simulink model "IEEE13_DVR_DSTATCOM_PV_Wind"  (R2022a)
settings: Solver=ode4  StartTime=0.0  StopTime=1.0  FixedStep=Ts  MaxStep=1e-4  RelTol=1e-4
InitFcn:
  | a=1; % Loading Factor
  | Ts=50e-6;
  | % phase to sequence conversion of RXB matrices
  | c=1*exp(sqrt(-1)*(120*pi/180));
  | T=[1 1 1;1 c*c c;1 c c*c];
  | Tinv=1/3*[1 1 1;1 c c*c;1 c*c c];
  | 
  | % Simulation data for the IEEE 13 Node Test Feeder model
  | mi2km = 1.60934;%  miles to km conversion
  | ft2km = 0.0003048; % feet to km conversion
  | ms2F = 1*1e-6/(2*pi*60);% microsiemens to Farads conversion
  | 
  | 
  | %% Configuration 601
  | % Series Resitance and Reactance - ohm/mile
  | R_601 = [0.3465 0.1560 0.1580;0.1560 0.3375 0.1535;0.1580 0.1535 0.3414];
  | X_601 = [1.1079 0.5017 0.4236;0.5017 1.0478 0.3849;0.4236 0.3849 1.0348];
  | % charging susceptance - microsiemens/mile
  | B_601 = [6.2998 -1.9958 -1.2595;-1.9958 5.9597 -0.7417;-1.2595 -0.7417 5.6386];
  | 
  | R_601 = R_601/mi2km;
  | Rseq=Tinv*R_601*T;
  | R1_601=Rseq(2,2);R0_601=Rseq(1,1);
  | 
  | L_601 = (X_601/(2*pi*60))/mi2km;
  | Lseq=Tinv*L_601*T;
  | L1_601=Lseq(2,2);L0_601=Lseq(1,1);
  | 
  | C_601 =(B_601*ms2F)/mi2km;
  | Cseq=Tinv*C_601*T;
  | C1_601=Cseq(2,2);C0_601=Cseq(1,1);
  | 
  | %% Configuration 602 - series reactance - ohm/mile
  | R_602 = [0.7526 0.1580 0.1560;0.1580 0.7475 0.1535;0.1560 0.1535 0.7436];
  | X_602 = [1.1814 0.4236 0.5017;0.4236 1.1983 0.3849;0.5017 0.3849 1.2112];
  | % charging susceptance - microsiemens/mile
  | B_602 = [5.6990 -1.0817 -1.6905;-1.0817 5.1795 -0.6588;-1.6905 -0.6588 5.4246];
  | 
  | R_602 = R_602/mi2km;
  | Rseq=Tinv*R_602*T;
  | R1_602=Rseq(2,2);R0_602=Rseq(1,1);
  | 
  | L_602 = (X_602/(2*pi*60))/mi2km;
  | Lseq=Tinv*L_602*T;
  | L1_602=Lseq(2,2);L0_602=Lseq(1,1);
  | 
  | C_602 =(B_602*ms2F)/mi2km;
  | Cseq=Tinv*C_602*T;
  | C1_602=Cseq(2,2);C0_602=Cseq(1,1);
  | %% Configuration 603 - series reactance - ohm/mile
  | R_603 = [0 0 0;0 1.3294 0.2066;0 0.2066 1.3238];
  | X_603 = [0 0 0;0 1.3471 0.4591;0 0.4591 1.3569];
  | % charging susceptance - microsiemens/mile
  | B_603 = [0 0 0;0 4.7097 -0.8999;0 -0.8999 4.6658];
  | 
  | % convert for SPS
  | R_603 = R_603/mi2km;
  | Rseq=Tinv*R_603*T;
  | R1_603=Rseq(2,2);R0_603=Rseq(1,1);
  | 
  | L_603 = (X_603/(2*pi*60))/mi2km;
  | Lseq=Tinv*L_603*T;
  | L1_603=Lseq(2,2);L0_603=Lseq(1,1);
  | 
  | C_603 =(B_603*ms2F)/mi2km;
  | Cseq=Tinv*C_603*T;
  | C1_603=Cseq(2,2);C0_603=Cseq(1,1);
  | %% Configuration 604 - series reactance - ohm/mile
  | R_604 = [1.3238 0 0.2066;0 0 0;0.2066 0 1.3294];
  | X_604 = [1.3569 0 0.4591;0 0 0;0.4591 0 1.3471];
  | % charging susceptance - microsiemens/mile
  | B_604 = [4.6658 0 -0.8999;0 0 0;-0.8999 0 4.7097];
  | R_604 = R_604/mi2km;
  | Rseq=Tinv*R_604*T;
  | R1_604=Rseq(2,2);R0_604=Rseq(1,1);
  | 
  | L_604 = (X_604/(2*pi*60))/mi2km;
  | Lseq=Tinv*L_604*T;
  | L1_604=Lseq(2,2);L0_604=Lseq(1,1);
  | 
  | C_604 =(B_604*ms2F)/mi2km;
  | Cseq=Tinv*C_604*T;
  | C1_604=Cseq(2,2);C0_604=Cseq(1,1);
  | %% Configuration 605 - series reactance - ohm/mile
  | R_605 = [0 0 0;0 0 0;0 0 1.3292];
  | X_605 = [0 0 0;0 0 0;0 0 1.3475];
  | % charging susceptance - microsiemens/mile
  | B_605 = [0 0 0;0 0 0;0 0 4.5193];
  | R_605 = R_605/mi2km;
  | Rseq=Tinv*R_605*T;
  | R1_605=Rseq(2,2);R0_605=Rseq(1,1);
  | 
  | L_605 = (X_605/(2*pi*60))/mi2km;
  | Lseq=Tinv*L_605*T;
  | L1_605=Lseq(2,2);L0_605=Lseq(1,1);
  | 
  | C_605 =(B_605*ms2F)/mi2km;
  | Cseq=Tinv*C_605*T;
  | C1_605=Cseq(2,2);C0_605=Cseq(1,1);
  | %% Configuration 606 - series reactance - ohm/mile
  | R_606 = [0.7982 0.3192 0.2849;0.3192 0.7891 0.3192;0.2849 0.3192 0.7982];
  | X_606 = [0.4463 0.0328 0.0143;0.0328 0.4041 0.0328;0.0143 0.0328 0.4463];
  | % charging susceptance - microsiemens/mile
  | B_606 = [96.8897 -1e-6 -1e-6;-1e-6 96.8897 -1e-6;-1e-6 -1e-6 96.8897];
  | R_606 = R_606/mi2km;
  | Rseq=Tinv*R_606*T;
  | R1_606=Rseq(2,2);R0_606=Rseq(1,1);
  | 
  | L_606 = (X_606/(2*pi*60))/mi2km;
  | Lseq=Tinv*L_606*T;
  | L1_606=Lseq(2,2);L0_606=Lseq(1,1);
  | 
  | C_606 =(B_606*ms2F)/mi2km;
  | Cseq=Tinv*C_606*T;
  | C1_606=Cseq(2,2);C0_606=Cseq(1,1);
  | %% Configuration 607 - series reactance - ohm/mile
  | R_607 = [1.3425 0 0;0 0 0;0 0 0];
  | X_607 = [0.5124 0 0;0 0 0;0 0 0];
  | % charging susceptance - microsiemens/mile
  | B_607 = [88.9912 0 0;0 0 0;0 0 0];
  | R_607 = R_607/mi2km;
  | Rseq=Tinv*R_607*T;
  | R1_607=Rseq(2,2);R0_607=Rseq(1,1);
  | 
  | L_607 = (X_607/(2*pi*60))/mi2km;
  | Lseq=Tinv*L_607*T;
  | L1_607=Lseq(2,2);L0_607=Lseq(1,1);
  | 
  | C_607 =(B_607*ms2F)/mi2km;
  | Cseq=Tinv*C_607*T;
  | C1_607=Cseq(2,2);C0_607=Cseq(1,1);
undefined symbols (not defined in the file): find_system
libraries: spsGroundLib x48, spsSeriesRLCBranchLib x46, spsThreePhaseVIMeasurementLib x19, spsControlledVoltageSourceLib x15, spsThreePhaseSeriesRLCLoadLib x7, spsRMSLib x7, spsThreePhaseBreakerLib x6, spsVoltageMeasurementLib x6, spsOnDelayLib x6, spsThreePhasePISectionLineLib x5, spsSeriesRLCLoadLib x5, spsMutualInductanceLib x4
(part 1 of 4)
settings Model: ARTEMISmethode_block_infos=$$__separator__$$pi34variableloadwith3PV/ARTEMIS Guide$$__separator__$$  Creator=Arun  LastModifiedBy=subas
settings SolverCC: ShapePreserveControl=EnableAll  AlgebraicLoopSolver=TrustRegion  SolverResetMethod=Robust
settings DataIOCC: ReturnWorkspaceOutputs=off
settings DebuggingCC: ArithmeticOperatorsInVariantConditions=warning
settings SFSimCC: SimUseLocalCustomCode=off  CustomCodeUndefinedFunction=UseInterfaceOnly
settings RTWCC: RTWUseLocalCustomCode=off
settings CodeAppCC: StateflowObjectComments=on
settings SimscapeCC: SimscapeNormalizeSystem=off

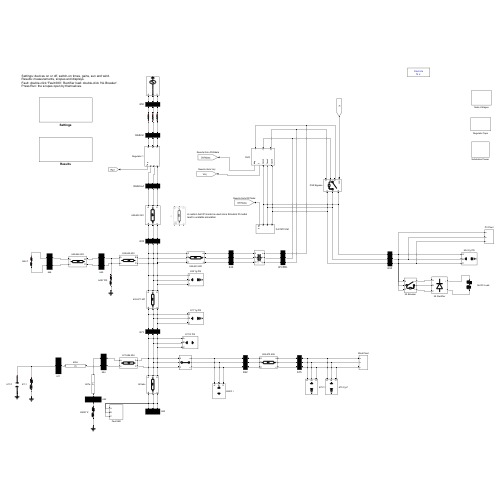
[thumbnail: Simulink's stored preview of the top-level diagram]
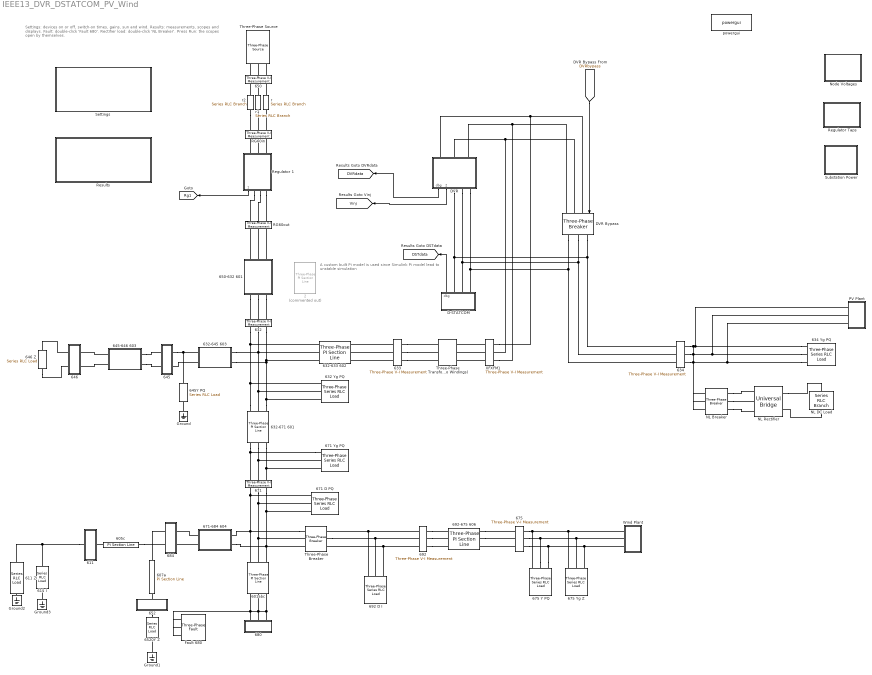
== system IEEE13_DVR_DSTATCOM_PV_Wind ==
  note: A custom built Pi model is used since Simulink Pi model
      | lead to unstable simulation
  note: Settings: devices on or off, switch-on times, gains, sun and wind.
      | Results: measurements, scopes and displays.
      | Fault: double-click 'Fault 680'. Rectifier load: double-click 'NL Breaker'.
      | Press Run: the scopes open by themselves.
  2 : spsThreePhasePISectionLineLib/Three-Phase PI Section Line  Commented=on  LConnTagsString=a|b|c  RConnTagsString=A|B|C  Length=2000*ft2km  Frequency=60  Resistances=[R1_601 R0_601]  Inductances=[L1_601 L0_601]  Capacitances=[C1_601 C0_601]
  601abc : spsThreePhasePISectionLineLib/Three-Phase PI Section Line  LConnTagsString=a|b|c  RConnTagsString=A|B|C  Length=1000*ft2km  Frequency=60  Resistances=[R1_601 R0_601]  Inductances=[L1_601 L0_601]  Capacitances=[C1_601 C0_601]
  605c : spsPiSectionLineLib/Pi Section Line  LConnTagsString=__new0  RConnTagsString=__new0  Phases=1  PiSections=1  Length=300*ft2km  Frequency=60  Resistance=R1_605  Inductance=L1_605  Capacitance=C1_605  SpecifyConductance=off  Conductance=0  Measurements=None  Measurements2=None
  607a : spsPiSectionLineLib/Pi Section Line  LConnTagsString=__new0  RConnTagsString=__new0  Phases=1  PiSections=1  Length=800*ft2km  Frequency=60  Resistance=R1_607  Inductance=L1_607  Capacitance=C1_607  SpecifyConductance=off  Conductance=0  Measurements=None  Measurements2=None
  611 : Subsystem
  611 I : spsSeriesRLCLoadLib/Series RLC Load  LConnTagsString=a  RConnTagsString=__new0  NominalVoltage=1*2401.78  NominalFrequency=60  ActivePower=170e3*a  InductivePower=80e3*a  CapacitivePower=0  Setx0=off  InitialVoltage=0  SetiL0=off  InitialCurrent=0  Measurements=None  LoadType=constant I
  611 Z : spsSeriesRLCLoadLib/Series RLC Load  LConnTagsString=a  RConnTagsString=__new0  NominalVoltage=2401.78  NominalFrequency=60  ActivePower=0  InductivePower=0  CapacitivePower=100e3*a  Setx0=off  InitialVoltage=0  SetiL0=off  InitialCurrent=0  Measurements=None  LoadType=constant Z
  632 : spsThreePhaseVIMeasurementLib/Three-Phase V-I Measurement  VoltageMeasurement=phase-to-ground  SetLabelV=on  LabelV=V632  Vpu=off  VpuLL=off  CurrentMeasurement=yes  SetLabelI=on  LabelI=I632  Ipu=off  Pbase=100e6  Vbase=24900  OutputType=Complex  PhasorSimulation=off  PSBequivalent=0
  632 Yg PQ : spsThreePhaseSeriesRLCLoadLib/Three-Phase Series RLC Load  LConnTagsString=A|B|C  Configuration=Y (grounded)  NominalVoltage=[ 1.021 1.042 1.0174]*2401.78  Vabc=[ 1 1 1]*2401.78  Vabcp=[1e3 1e3 1e3]  NominalFrequency=60  UnbalancedPower=on  ActivePower="[17 66  117]*1e3/2"  InductivePower="[10 38  68]*1e3/2"  CapacitivePower=100  Pabc="[17 66  117]*1e3/2*a"  QLabc="[10 38  68]*1e3/2*a"  QCabc=[0 0 0]  Pabcp=[10e3 9e3 11e3]  QLabcp=[100 90 110]  QCabcp=[100 90 110]  Measurements=None  LoadType=constant PQ
  632-633 602 : spsThreePhasePISectionLineLib/Three-Phase PI Section Line  LConnTagsString=a|b|c  RConnTagsString=A|B|C  Length=500*ft2km  Frequency=60  Resistances=[R1_602 R0_602]  Inductances=[L1_602 L0_602]  Capacitances=[C1_602 C0_602]
  632-645 603 : Subsystem  mask(Two-Phase PI Section Block){Rl=R_603, Ll=L_603, Cl=C_603, L=500*ft2km}
      mask prompts: Rl "Resistance per unit Length(Ohm/Km)[3x3 matrix]"; Ll "Inductance per unit Length(H/Km)[3x3 matrix]"; Cl "Capacitance per unit Length(F/Km)[3x3 matrix"; L "Length (Km)"
      mask help: This block models a two-phase transmission line with a single PI section.
      mask init:
      | W = sign(sum(abs(Rl)));
      | s = find(W==1);%Identify non zero rows and columns
      | 
      | Rt =Rl(s,s);
      | Rl= Rt;
      | Lt =Ll(s,s);
      | Ll= Lt;
      | Ct =Cl(s,s);
      | Cl= Ct;
      mask Display:
      | color('black')
      | plot(0,0,100,100,[20,20,80,80,90,80,80,20,20,10],[50,40,40,50,50,50,61,61,50,50],[56,39],[55,55],[44,44],[44,55],[53,50,50],[44,48,55])
      | color('black')
      | port_label('RConn', 1, 'b')
      | port_label('RConn', 2, 'c')
      | port_label('LConn', 1, 'B')
      | port_label('LConn', 2, 'C')
  632-671 601 : spsThreePhasePISectionLineLib/Three-Phase PI Section Line  LConnTagsString=a|b|c  RConnTagsString=A|B|C  Length=2000*ft2km  Frequency=60  Resistances=[R1_601 R0_601]  Inductances=[L1_601 L0_601]  Capacitances=[C1_601 C0_601]
  633 : spsThreePhaseVIMeasurementLib/Three-Phase V-I Measurement  VoltageMeasurement=phase-to-ground  SetLabelV=on  LabelV=V633  Vpu=off  VpuLL=off  CurrentMeasurement=no  SetLabelI=on  LabelI=I634  Ipu=off  Pbase=100e6  Vbase=24900  OutputType=Complex  PhasorSimulation=off  PSBequivalent=0
  634 : spsThreePhaseVIMeasurementLib/Three-Phase V-I Measurement  VoltageMeasurement=phase-to-ground  SetLabelV=on  LabelV=V634  Vpu=off  VpuLL=off  CurrentMeasurement=yes  SetLabelI=on  LabelI=I634  Ipu=off  Pbase=100e6  Vbase=24900  OutputType=Complex  PhasorSimulation=off  PSBequivalent=0
  634 Yg PQ : spsThreePhaseSeriesRLCLoadLib/Three-Phase Series RLC Load  LConnTagsString=A|B|C  Configuration=Y (grounded)  NominalVoltage=[ 1.021 1.042 1.0174]*2401.78  Vabc=[1 1 1]*277.128  Vabcp=[1e3 1e3 1e3]  NominalFrequency=60  UnbalancedPower=on  ActivePower="[17 66  117]*1e3/2"  InductivePower="[10 38  68]*1e3/2"  CapacitivePower=100  Pabc=[160 120 120]*1e3*a  QLabc=[110 90 90]*1e3*a  QCabc=[0 0 0]  Pabcp=[10e3 9e3 11e3]  QLabcp=[100 90 110]  QCabcp=[100 90 110]  Measurements=None  LoadType=constant PQ
  645 : Subsystem
  645-646 603 : Subsystem  mask(Two-Phase PI Section Block){Rl=R_603, Ll=L_603, Cl=C_603, L=300*ft2km}
      mask prompts: Rl "Resistance per unit Length(Ohm/Km)[3x3 matrix]"; Ll "Inductance per unit Length(H/Km)[3x3 matrix]"; Cl "Capacitance per unit Length(F/Km)[3x3 matrix"; L "Length (Km)"
      mask help: This block models a two-phase transmission line with a single PI section.
      mask init:
      | W = sign(sum(abs(Rl)));
      | s = find(W==1);%Identify non zero rows and columns
      | 
      | Rt =Rl(s,s);
      | Rl= Rt;
      | Lt =Ll(s,s);
      | Ll= Lt;
      | Ct =Cl(s,s);
      | Cl= Ct;
      mask Display:
      | color('black')
      | plot(0,0,100,100,[20,20,80,80,90,80,80,20,20,10],[50,40,40,50,50,50,61,61,50,50],[56,39],[55,55],[44,44],[44,55],[53,50,50],[44,48,55])
      | color('black')
      | port_label('RConn', 1, 'b')
      | port_label('RConn', 2, 'c')
      | port_label('LConn', 1, 'B')
      | port_label('LConn', 2, 'C')
  645Y PQ : spsSeriesRLCLoadLib/Series RLC Load  LConnTagsString=a  RConnTagsString=__new0  NominalVoltage=1*2401.78  NominalFrequency=60  ActivePower=170e3*a  InductivePower=125e3*a  CapacitivePower=0  Setx0=off  InitialVoltage=0  SetiL0=off  InitialCurrent=0  Measurements=None  LoadType=constant PQ
  646 : Subsystem
  646 Z : spsSeriesRLCLoadLib/Series RLC Load  LConnTagsString=a  RConnTagsString=__new0  NominalVoltage=4160  NominalFrequency=60  ActivePower=230e3*a  InductivePower=132e3*a  CapacitivePower=0  Setx0=off  InitialVoltage=0  SetiL0=off  InitialCurrent=0  Measurements=None  LoadType=constant Z
  650 : spsThreePhaseVIMeasurementLib/Three-Phase V-I Measurement  VoltageMeasurement=phase-to-ground  SetLabelV=on  LabelV=V650  Vpu=off  VpuLL=off  CurrentMeasurement=yes  SetLabelI=on  LabelI=I650  Ipu=off  Pbase=100e6  Vbase=24900  OutputType=Complex  PhasorSimulation=off  PSBequivalent=0
  650-632 601 : Subsystem  mask(Three-Phase PI Section Block){Rl=R_601, Ll=L_601, Cl=C_601, L=2000*ft2km}
      mask prompts: Rl "Resistance per unit Length(Ohm/Km)[3x3 matrix]"; Ll "Inductance per unit Length(H/Km)[3x3 matrix]"; Cl "Capacitance per unit Length(F/Km)[3x3 matrix]"; L "Length (Km)"
      mask help: This block models a three-phase transmission line with a single PI section.
      mask Display:
      | color('black')
      | plot(0,0,100,100,[20,20,80,80,90,80,80,20,20,10],[50,40,40,50,50,50,61,61,50,50],[56,39],[55,55],[44,44],[44,55],[53,50,50],[44,48,55])
      | color('black')
      | port_label('RConn', 1, 'a')
      | port_label('RConn', 2, 'b')
      | port_label('RConn', 3, 'c')
      | port_label('LConn', 1, 'A')
      | port_label('LConn', 2, 'B')
      | port_label('LConn', 3, 'C')
  652 : Subsystem
  6520Y Z : spsSeriesRLCLoadLib/Series RLC Load  LConnTagsString=a  RConnTagsString=__new0  NominalVoltage=1.0*2401.78  NominalFrequency=60  ActivePower=128e3*a  InductivePower=86e3*a  CapacitivePower=0  Setx0=off  InitialVoltage=0  SetiL0=off  InitialCurrent=0  Measurements=None  LoadType=constant Z
  671 : spsThreePhaseVIMeasurementLib/Three-Phase V-I Measurement  VoltageMeasurement=phase-to-ground  SetLabelV=on  LabelV=V671  Vpu=off  VpuLL=off  CurrentMeasurement=no  SetLabelI=on  LabelI=I634  Ipu=off  Pbase=100e6  Vbase=24900  OutputType=Complex  PhasorSimulation=off  PSBequivalent=0
  671 D PQ : spsThreePhaseSeriesRLCLoadLib/Three-Phase Series RLC Load  LConnTagsString=A|B|C  Configuration=Delta  NominalVoltage=[ 1.021 1.042 1.0174]*2401.78  Vabc=[ 1.73773 1.77224 1.71484]*2401.78  Vabcp=[ 1 1 1]*4160  NominalFrequency=60  UnbalancedPower=on  ActivePower="[17 66  117]*1e3/2"  InductivePower="[10 38  68]*1e3/2"  CapacitivePower=100  Pabc=[385 385 385 ]*1e3  QLabc=[220 220 220]*1e3  QCabc=[0 0 0]  Pabcp=[385 385 385 ]*1e3*a  QLabcp=[220 220 220]*1e3*a  QCabcp="[0  0  0]"  Measurements=Branch voltages and currents  LoadType=constant PQ
  671 Yg PQ : spsThreePhaseSeriesRLCLoadLib/Three-Phase Series RLC Load  LConnTagsString=A|B|C  Configuration=Y (grounded)  NominalVoltage=[ 1.021 1.042 1.0174]*2401.78  Vabc=[ 1 1 1]*2401.78  Vabcp=[1e3 1e3 1e3]  NominalFrequency=60  UnbalancedPower=on  ActivePower="[17 66  117]*1e3/2"  InductivePower="[10 38  68]*1e3/2"  CapacitivePower=100  Pabc="[17 66  117]*1e3/2*a"  QLabc="[10 38  68]*1e3/2*a"  QCabc=[0 0 0]  Pabcp=[10e3 9e3 11e3]  QLabcp=[100 90 110]  QCabcp=[100 90 110]  Measurements=None  LoadType=constant PQ
  671-684 604 : Subsystem  mask(Two-Phase PI Section Block){Rl=R_604, Ll=L_604, Cl=C_604, L=300*ft2km}
      mask prompts: Rl "Resistance per unit Length(Ohm/Km)[3x3 matrix]"; Ll "Inductance per unit Length(H/Km)[3x3 matrix]"; Cl "Capacitance per unit Length(F/Km)[3x3 matrix"; L "Length (Km)"
      mask help: This block models a two-phase transmission line with a single PI section.
      mask init:
      | W = sign(sum(abs(Rl)));
      | s = find(W==1);%Identify non zero rows and columns
      | 
      | Rt =Rl(s,s);
      | Rl= Rt;
      | Lt =Ll(s,s);
      | Ll= Lt;
      | Ct =Cl(s,s);
      | Cl= Ct;
      mask Display:
      | color('black')
      | plot(0,0,100,100,[20,20,80,80,90,80,80,20,20,10],[50,40,40,50,50,50,61,61,50,50],[56,39],[55,55],[44,44],[44,55],[53,50,50],[44,48,55])
      | color('black')
      | port_label('RConn', 1, 'a')
      | port_label('RConn', 2, 'c')
      | port_label('LConn', 1, 'A')
      | port_label('LConn', 2, 'C')
  675 : spsThreePhaseVIMeasurementLib/Three-Phase V-I Measurement  VoltageMeasurement=phase-to-ground  SetLabelV=on  LabelV=V675  Vpu=off  VpuLL=off  CurrentMeasurement=no  SetLabelI=on  LabelI=I634  Ipu=off  Pbase=100e6  Vbase=24900  OutputType=Complex  PhasorSimulation=off  PSBequivalent=0
  675 Y PQ : spsThreePhaseSeriesRLCLoadLib/Three-Phase Series RLC Load  LConnTagsString=A|B|C  Configuration=Y (grounded)  NominalVoltage=[ 1.021 1.042 1.0174]*2401.78  Vabc=[ 1 1 1]*2401.78  Vabcp=[1e3 1e3 1e3]  NominalFrequency=60  UnbalancedPower=on  ActivePower="[17 66  117]*1e3/2"  InductivePower="[10 38  68]*1e3/2"  CapacitivePower=100  Pabc="[485  68  290]*1e3*a"  QLabc="[190  60  212]*1e3*a"  QCabc=[0 0 0]  Pabcp=[10e3 9e3 11e3]  QLabcp=[100 90 110]  QCabcp=[100 90 110]  Measurements=Branch voltages and currents  LoadType=constant PQ
  675 Yg Z : spsThreePhaseSeriesRLCLoadLib/Three-Phase Series RLC Load  LConnTagsString=A|B|C  Configuration=Y (grounded)  NominalVoltage=[ 1.021 1.042 1.0174]*2401.78  Vabc=[ 1.0 1.0 1.0]*2401.78  Vabcp=[1e3 1e3 1e3]  NominalFrequency=60  UnbalancedPower=on  ActivePower="[17 66  117]*1e3/2"  InductivePower="[10 38  68]*1e3/2"  CapacitivePower=100  Pabc=[0 0 0]  QLabc=[0 0 0]  QCabc=[200 200 200]*1e3*a  Pabcp=[10e3 9e3 11e3]  QLabcp=[100 90 110]  QCabcp=[100 90 110]  Measurements=None  LoadType=constant Z
  680 : Subsystem
  684 : Subsystem
  692 : spsThreePhaseVIMeasurementLib/Three-Phase V-I Measurement  VoltageMeasurement=phase-to-ground  SetLabelV=on  LabelV=V692  Vpu=off  VpuLL=off  CurrentMeasurement=no  SetLabelI=on  LabelI=I634  Ipu=off  Pbase=100e6  Vbase=24900  OutputType=Complex  PhasorSimulation=off  PSBequivalent=0
  692 D I : spsThreePhaseSeriesRLCLoadLib/Three-Phase Series RLC Load  LConnTagsString=A|B|C  Configuration=Delta  NominalVoltage=[ 1.021 1.042 1.0174]*2401.78  Vabc=[ 1.73488 1.75203 1.72341]*2401.78  Vabcp=[ 1.0 1.0 1.0]*4160  NominalFrequency=60  UnbalancedPower=on  ActivePower="[17 66  117]*1e3/2"  InductivePower="[10 38  68]*1e3/2"  CapacitivePower=100  Pabc="[17 66  117]*1e3/2"  QLabc="[10 38  68]*1e3/2"  QCabc=[0 0 0]  Pabcp=[1e-3 1e-3 170 ]*1e3*a  QLabcp=[0 0 151]*1e3*a  QCabcp="[0  0  0]"  Measurements=Branch voltages and currents  LoadType=constant Z
  692-675 606 : spsThreePhasePISectionLineLib/Three-Phase PI Section Line  LConnTagsString=a|b|c  RConnTagsString=A|B|C  Length=500*ft2km  Frequency=60  Resistances=[R1_606 R0_606]  Inductances=[L1_606 L0_606]  Capacitances=[C1_606 C0_606]
  D-STATCOM : Subsystem
  DVR : Subsystem
  DVR Bypass : spsThreePhaseBreakerLib/Three-Phase Breaker  InitialState=open  SwitchA=on  SwitchB=on  SwitchC=on  SwitchTimes="[1/60  5/60]"  External=on  BreakerResistance=1e-3  SnubberResistance=1e6  SnubberCapacitance=inf  Measurements=None
  Fault 680 : spsThreePhaseFaultLib/Three-Phase Fault  InitialStates=0  FaultA=on  FaultB=off  FaultC=off  GroundFault=on  SwitchTimes=[0.6 0.8]  External=off  SwitchStatus=NaN  FaultResistance=0.01  GroundResistance=0.01  SnubberResistance=1e6  SnubberCapacitance=inf  Measurements=None
  Ground{,1..3} (4 alike) : spsGroundLib/Ground  LConnTagsString=a
  NL Breaker : spsThreePhaseBreakerLib/Three-Phase Breaker  InitialState=open  SwitchA=on  SwitchB=on  SwitchC=on  SwitchTimes=[0.3]  External=off  BreakerResistance=0.01  SnubberResistance=1e6  SnubberCapacitance=inf  Measurements=None
  NL DC Load : spsSeriesRLCBranchLib/Series RLC Branch  LConnTagsString=__new0  RConnTagsString=__new0  BranchType=RL  Resistance=4.2  Inductance=5e-3  SetiL0=off  InitialCurrent=0  Capacitance=1e-6  Setx0=off  InitialVoltage=0  Measurements=None
  NL Rectifier : spsUniversalBridgeLib/Universal Bridge  Arms=3  SnubberResistance=1e5  SnubberCapacitance=inf  Device=Diodes  Ron=1e-3  Lon=0  ForwardVoltages="[  0  0  ]"  ForwardVoltage=0  GTOparameters=[ 10e-6 , 20e-6 ]  IGBTparameters=[ 1e-6 , 2e-6 ]  Measurements=None  Measurements_2=None  converterType=Rectifier
  Node Voltages : Subsystem
  PV Plant : Subsystem
  RG60in : spsThreePhaseVIMeasurementLib/Three-Phase V-I Measurement  VoltageMeasurement=phase-to-ground  SetLabelV=on  LabelV=RG60in  Vpu=off  VpuLL=off  CurrentMeasurement=yes  SetLabelI=on  LabelI=IRG60in  Ipu=off  Pbase=100e6  Vbase=24900  OutputType=Complex  PhasorSimulation=off  PSBequivalent=0
  RG60out : spsThreePhaseVIMeasurementLib/Three-Phase V-I Measurement  VoltageMeasurement=phase-to-ground  SetLabelV=on  LabelV=RG60out  Vpu=off  VpuLL=off  CurrentMeasurement=yes  SetLabelI=on  LabelI=IRG60out  Ipu=off  Pbase=100e6  Vbase=24900  OutputType=Complex  PhasorSimulation=off  PSBequivalent=0
  Regulator 1 : Subsystem
  "Regulator Taps " : Subsystem
  Results : Subsystem
  Settings : Subsystem
  Substation Power : Subsystem
  Three-Phase Transformer (Two Windings) : spsThreePhaseTransformerTwoWindingsLib/Three-Phase Transformer (Two Windings)  Winding1Connection=Yg  Winding2Connection=Yg  CoreType=Three single-phase transformers  SetSaturation=off  Hysteresis=off  DataFile='hysteresis'  SetInitialFlux=off  Measurements=None  UNITS=pu  NominalPower=[ 500e3 , 60 ]  Winding1=[4160 0.011 0.02]  Winding2=[480 0 0]  Rm=500  Lm=500  L0=0.5  Saturation=[ 0,0 ; 0.0024,1.2 ; 1.0,1.52 ]  InitialFluxes=[ 0.8 , -0.8 , 0.7 ]  BreakLoop=off  DiscreteSolver=Trapezoidal iterative  DataType=off  TransfoNumber=1
  Three-Phase Breaker : spsThreePhaseBreakerLib/Three-Phase Breaker  InitialState=closed  SwitchA=off  SwitchB=off  SwitchC=off  SwitchTimes=[0.5 ]  External=off  BreakerResistance=0.0001  SnubberResistance=inf  SnubberCapacitance=0  Measurements=None
  Three-Phase Source : spsThreePhaseSourceLib/Three-Phase Source  InternalConnection=Yg  VoltagePhases=on  Voltage=25e3  PhaseAngle=0  Voltage_phases=[ 1.0 1.0 1.0]*2401.78  PhaseAngles_phases=[0 -120 120]  Frequency=60  NonIdealSource=off  SpecifyImpedance=off  Resistance=.001  Inductance=16.58e-6  ShortCircuitLevel=100e6  BaseVoltage=4160  XRratio=7  BusType=swing  Pref=10e3  Qref=0  Prefabc=[10e3, 10e3, 10e3]  Qrefabc=[0, 0, 0]  Qmin=-inf  Qmax=inf
  Wind Plant : Subsystem
  XFXFM1 : spsThreePhaseVIMeasurementLib/Three-Phase V-I Measurement  VoltageMeasurement=phase-to-ground  SetLabelV=on  LabelV=XFXFM1  Vpu=off  VpuLL=off  CurrentMeasurement=yes  SetLabelI=on  LabelI=Is634  Ipu=off  Pbase=100e6  Vbase=24900  OutputType=Complex  PhasorSimulation=off  PSBequivalent=0
  powergui : spspowerguiLib/powergui  Priority=1  SimulationMode=Discrete  SampleTime=Ts  frequency=60  Iterations=50  frequencyindice=0  Pbase=100e6  ErrMax=1e-4  UnitsV=kV  UnitsW=MW  buscounter=0  FunctionMessages=off  echomessages=on  EnableUseOfTLC=off  CurrentSourceSwitches=off  DisableSnubberDevices=off  DisableRonSwitches=off  DisableVfSwitches=off  DisplayEquations=off  AutomaticDiscreteSolvers=off  SolverType=Tustin/Backward Euler (TBE)  Interpol=off  ExternalGateDelay=off  methode=off  Ts=0  x0status=blocks  SPID=off  SwTol=0  HookPort=off  NonlinearTolerance=1e-4  nMaxIteration=100  ContinueOnMaxIteration=off  RestoreLinks=warning  ResistiveCurrentMeasurement=off  Frange=[0:2:500]  Ylog=off  Xlog=on  ShowGrid=off  save=off  variable=ZData  structure=0  ZoomFFT=off  StartTime=0.0  cycles=1  DisplayStyle=1  fundamental=60  FreqAxis=off  MaxFrequency=1000  frequencyindicesteady=1  RmsSteady=1  display=off
  r : spsSeriesRLCBranchLib/Series RLC Branch  LConnTagsString=__new0  RConnTagsString=__new0  BranchType=R  Resistance=1e-6  Inductance=1e-6  SetiL0=off  InitialCurrent=0  Capacitance=1e-6  Setx0=off  InitialVoltage=0  Measurements=None
  r1 : spsSeriesRLCBranchLib/Series RLC Branch  LConnTagsString=__new0  RConnTagsString=__new0  BranchType=R  Resistance=1e-6  Inductance=1e-6  SetiL0=off  InitialCurrent=0  Capacitance=1e-6  Setx0=off  InitialVoltage=0  Measurements=None
  r2 : spsSeriesRLCBranchLib/Series RLC Branch  LConnTagsString=__new0  RConnTagsString=__new0  BranchType=R  Resistance=1e-6  Inductance=1e-6  SetiL0=off  InitialCurrent=0  Capacitance=1e-6  Setx0=off  InitialVoltage=0  Measurements=None
  tag scope: DSTdata=global, DVRdata=global, Rg1=global, Vinj=global
  wires:
  Regulator 1/1(Tap) -> [Rg1]
  DVR/1(dbg) -> [DVRdata]
  DVR/2(Out2) -> [Vinj]
  D-STATCOM/1(dbg) -> [DSTdata]
  [DVRbypass] -> DVR Bypass/1
  connections:
  632-645 603/LConn1 -- 632 Yg PQ/LConn2 -- 632-671 601/LConn2 -- 632-633 602/LConn2 -- 632/RConn2
  Three-Phase Breaker/LConn1 -- 671 D PQ/LConn1 -- 671/RConn1 -- 601abc/LConn1 -- 671-684 604/LConn1
  611/LConn1 -- 611 Z/LConn1 -- 611 I/LConn1
  675 Y PQ/LConn2 -- 675 Yg Z/LConn2 -- Wind Plant/RConn2 -- 675/RConn2
  671 Yg PQ/LConn1 -- 671/LConn1 -- 632-671 601/RConn1
  632-671 601/LConn3 -- 632 Yg PQ/LConn3 -- 632/RConn3 -- 632-633 602/LConn3 -- 632-645 603/LConn2
  601abc/LConn2 -- Three-Phase Breaker/LConn2 -- 671 D PQ/LConn2 -- 671/RConn2
  645/RConn1 -- 632-645 603/RConn1 -- 645Y PQ/LConn1
  692/LConn1 -- 692 D I/LConn1 -- Three-Phase Breaker/RConn1
  Wind Plant/RConn1 -- 675 Yg Z/LConn1 -- 675/RConn1 -- 675 Y PQ/LConn1
  671/LConn3 -- 632-671 601/RConn3 -- 671 Yg PQ/LConn3
  671/LConn2 -- 632-671 601/RConn2 -- 671 Yg PQ/LConn2
  632-671 601/LConn1 -- 632 Yg PQ/LConn1 -- 632/RConn1 -- 632-633 602/LConn1
  692/LConn3 -- 692 D I/LConn3 -- Three-Phase Breaker/RConn3
  671-684 604/LConn2 -- 671 D PQ/LConn3 -- 671/RConn3 -- 601abc/LConn3 -- Three-Phase Breaker/LConn3
  675 Y PQ/LConn3 -- 675 Yg Z/LConn3 -- Wind Plant/RConn3 -- 675/RConn3
  692/LConn2 -- 692 D I/LConn2 -- Three-Phase Breaker/RConn2
  684/LConn1 -- 607a/LConn1
  r1/RConn1 -- RG60in/LConn2
  r/RConn1 -- RG60in/LConn3
  645-646 603/RConn2 -- 646/RConn2
  601abc/RConn1 -- 680/RConn1 -- Fault 680/LConn1
  605c/LConn1 -- 684/LConn2
  692/RConn2 -- 692-675 606/LConn2
  646 Z/RConn1 -- 646/LConn2
  650-632 601/RConn1 -- 632/LConn1
  r1/LConn1 -- 650/RConn2
  692-675 606/RConn1 -- 675/LConn1
  675/LConn3 -- 692-675 606/RConn3
  Regulator 1/LConn3 -- RG60in/RConn3
  650-632 601/RConn3 -- 632/LConn3
  652/LConn1 -- 6520Y Z/LConn1
  Ground1/LConn1 -- 6520Y Z/RConn1
  633/LConn1 -- 632-633 602/RConn1
  Regulator 1/RConn2 -- RG60out/LConn2
  633/LConn3 -- 632-633 602/RConn3
  605c/RConn1 -- 611/RConn1
  XFXFM1/LConn2 -- Three-Phase Transformer (Two Windings)/RConn2
  601abc/RConn3 -- 680/RConn3 -- Fault 680/LConn3
  633/RConn2 -- Three-Phase Transformer (Two Windings)/LConn2
  634 Yg PQ/LConn2 -- 634/RConn2 -- NL Breaker/LConn2 -- PV Plant/RConn2
  Ground3/LConn1 -- 611 I/RConn1
  601abc/RConn2 -- 680/RConn2 -- Fault 680/LConn2
  r/LConn1 -- 650/RConn3
  Regulator 1/LConn1 -- RG60in/RConn1
  Regulator 1/RConn3 -- RG60out/LConn3
  Ground/LConn1 -- 645Y PQ/RConn1
  632-645 603/RConn2 -- 645/RConn2
  633/RConn3 -- Three-Phase Transformer (Two Windings)/LConn3
  634 Yg PQ/LConn3 -- 634/RConn3 -- NL Breaker/LConn3 -- PV Plant/RConn3
  r2/RConn1 -- RG60in/LConn1
  692/RConn1 -- 692-675 606/LConn1
  633/RConn1 -- Three-Phase Transformer (Two Windings)/LConn1
  650/LConn3 -- Three-Phase Source/RConn3
  Regulator 1/LConn2 -- RG60in/RConn2
  633/LConn2 -- 632-633 602/RConn2
  645-646 603/RConn1 -- 646/RConn1
  671-684 604/RConn2 -- 684/RConn2
  692/RConn3 -- 692-675 606/LConn3
  652/RConn1 -- 607a/RConn1
  645-646 603/LConn1 -- 645/LConn1
  650-632 601/LConn3 -- RG60out/RConn3
  650-632 601/LConn2 -- RG60out/RConn2
  650/LConn2 -- Three-Phase Source/RConn2
  XFXFM1/LConn3 -- Three-Phase Transformer (Two Windings)/RConn3
  Ground2/LConn1 -- 611 Z/RConn1
  671-684 604/RConn1 -- 684/RConn1
  Regulator 1/RConn1 -- RG60out/LConn1
  692-675 606/RConn2 -- 675/LConn2
  r2/LConn1 -- 650/RConn1
  646/LConn1 -- 646 Z/LConn1
  645-646 603/LConn2 -- 645/LConn2
  XFXFM1/LConn1 -- Three-Phase Transformer (Two Windings)/RConn1
  650/LConn1 -- Three-Phase Source/RConn1
  650-632 601/RConn2 -- 632/LConn2
  650-632 601/LConn1 -- RG60out/RConn1
  NL Breaker/RConn1 -- NL Rectifier/LConn1
  NL Breaker/RConn2 -- NL Rectifier/LConn2
  NL Breaker/RConn3 -- NL Rectifier/LConn3
  NL Rectifier/RConn1 -- NL DC Load/LConn1
  NL DC Load/RConn1 -- NL Rectifier/RConn2
  XFXFM1/RConn1 -- DVR/LConn1 -- DVR Bypass/LConn1
  DVR/RConn1 -- DVR Bypass/RConn1 -- 634/LConn1 -- D-STATCOM/RConn1
  DVR Bypass/LConn2 -- DVR/LConn2 -- XFXFM1/RConn2
  DVR/RConn2 -- D-STATCOM/RConn2 -- DVR Bypass/RConn2 -- 634/LConn2
  XFXFM1/RConn3 -- DVR Bypass/LConn3 -- DVR/LConn3
  DVR/RConn3 -- D-STATCOM/RConn3 -- DVR Bypass/RConn3 -- 634/LConn3
  634 Yg PQ/LConn1 -- 634/RConn1 -- NL Breaker/LConn1 -- PV Plant/RConn1

== system IEEE13_DVR_DSTATCOM_PV_Wind/611 ==
  1 : spsThreePhaseVIMeasurementLib/Three-Phase V-I Measurement  VoltageMeasurement=phase-to-ground  SetLabelV=on  LabelV=V611  Vpu=off  VpuLL=off  CurrentMeasurement=no  SetLabelI=on  LabelI=I634  Ipu=off  Pbase=100e6  Vbase=24900  OutputType=Complex  PhasorSimulation=off  PSBequivalent=0
  Ground{1..2,9,12} (4 alike) : spsGroundLib/Ground  LConnTagsString=a
  c : PMIOPort  Side=Left
  C : PMIOPort  Port=2  Side=Right
  connections:
  Ground12/LConn1 -- 1/LConn2
  Ground9/LConn1 -- 1/RConn2
  1/LConn3 -- C/RConn1
  1/RConn3 -- c/RConn1
  Ground1/LConn1 -- 1/RConn1
  Ground2/LConn1 -- 1/LConn1

== system IEEE13_DVR_DSTATCOM_PV_Wind/632-645 603 ==
  Config300 : spsMutualInductanceLib/Mutual Inductance  LConnTagsString=a|b  RConnTagsString=A|B  TypeOfMutual=Generalized mutual inductance  NumberOfWindings=2  SelfImpedance1=[1.1 1.1e-03]  SelfImpedance2=[ 1.1 1.1e-03]  ThreeWindings=on  SelfImpedance3=[ 1.1 1.1e-03]  MutualImpedance=[1.0 1.0e-03]  InductanceMatrix=Ll* L  ResistanceMatrix=Rl* L  Measurements=None
  Ground{2..3,5..6} (4 alike) : spsGroundLib/Ground  LConnTagsString=a
  Series RLC Branch : spsSeriesRLCBranchLib/Series RLC Branch  LConnTagsString=__new0  RConnTagsString=__new0  BranchType=C  Resistance=1  Inductance=1e-3  SetiL0=off  InitialCurrent=0  Capacitance=Cl(1,2)/2*L  Setx0=off  InitialVoltage=0  Measurements=None
  Series RLC Branch1 : spsSeriesRLCBranchLib/Series RLC Branch  LConnTagsString=__new0  RConnTagsString=__new0  BranchType=C  Resistance=1  Inductance=1e-3  SetiL0=off  InitialCurrent=0  Capacitance=Cl(1,2)/2*L  Setx0=off  InitialVoltage=0  Measurements=None
  Series RLC Branch11 : spsSeriesRLCBranchLib/Series RLC Branch  LConnTagsString=__new0  RConnTagsString=__new0  BranchType=C  Resistance=1  Inductance=1e-3  SetiL0=off  InitialCurrent=0  Capacitance=Cl(1,1)/2*L  Setx0=off  InitialVoltage=0  Measurements=None
  Series RLC Branch2 : spsSeriesRLCBranchLib/Series RLC Branch  LConnTagsString=__new0  RConnTagsString=__new0  BranchType=C  Resistance=1  Inductance=1e-3  SetiL0=off  InitialCurrent=0  Capacitance=Cl(1,1)/2*L  Setx0=off  InitialVoltage=0  Measurements=None
  Series RLC Branch3 : spsSeriesRLCBranchLib/Series RLC Branch  LConnTagsString=__new0  RConnTagsString=__new0  BranchType=C  Resistance=1  Inductance=1e-3  SetiL0=off  InitialCurrent=0  Capacitance=Cl(2,2)/2*L  Setx0=off  InitialVoltage=0  Measurements=None
  Series RLC Branch9 : spsSeriesRLCBranchLib/Series RLC Branch  LConnTagsString=__new0  RConnTagsString=__new0  BranchType=C  Resistance=1  Inductance=1e-3  SetiL0=off  InitialCurrent=0  Capacitance=Cl(2,2)/2*L  Setx0=off  InitialVoltage=0  Measurements=None
  B In : PMIOPort  Side=Left
  C in : PMIOPort  Port=2  Side=Left
  B Out : PMIOPort  Port=3  Side=Right
  C Out : PMIOPort  Port=4  Side=Right
  connections:
  Config300/LConn1 -- Series RLC Branch/LConn1 -- B In/RConn1 -- Series RLC Branch11/LConn1
  Config300/RConn1 -- Series RLC Branch2/LConn1 -- Series RLC Branch1/LConn1 -- B Out/RConn1
  Config300/LConn2 -- Series RLC Branch9/LConn1 -- Series RLC Branch/RConn1 -- C in/RConn1
  Config300/RConn2 -- Series RLC Branch3/LConn1 -- Series RLC Branch1/RConn1 -- C Out/RConn1
  Ground3/LConn1 -- Series RLC Branch11/RConn1
  Ground6/LConn1 -- Series RLC Branch9/RConn1
  Series RLC Branch3/RConn1 -- Ground5/LConn1
  Series RLC Branch2/RConn1 -- Ground2/LConn1

== system IEEE13_DVR_DSTATCOM_PV_Wind/645 ==
  1 : spsThreePhaseVIMeasurementLib/Three-Phase V-I Measurement  VoltageMeasurement=phase-to-ground  SetLabelV=on  LabelV=V645  Vpu=off  VpuLL=off  CurrentMeasurement=no  SetLabelI=on  LabelI=I634  Ipu=off  Pbase=100e6  Vbase=24900  OutputType=Complex  PhasorSimulation=off  PSBequivalent=0
  Ground12 : spsGroundLib/Ground  LConnTagsString=a
  Ground9 : spsGroundLib/Ground  LConnTagsString=a
  B : PMIOPort  Side=Right
  b : PMIOPort  Port=2  Side=Left
  c : PMIOPort  Port=3  Side=Left
  C : PMIOPort  Port=4  Side=Right
  connections:
  Ground12/LConn1 -- 1/LConn1
  1/LConn3 -- C/RConn1
  1/LConn2 -- B/RConn1
  Ground9/LConn1 -- 1/RConn1
  1/RConn2 -- b/RConn1
  1/RConn3 -- c/RConn1

== system IEEE13_DVR_DSTATCOM_PV_Wind/645-646 603 ==
  Config300 : spsMutualInductanceLib/Mutual Inductance  LConnTagsString=a|b  RConnTagsString=A|B  TypeOfMutual=Generalized mutual inductance  NumberOfWindings=2  SelfImpedance1=[1.1 1.1e-03]  SelfImpedance2=[ 1.1 1.1e-03]  ThreeWindings=on  SelfImpedance3=[ 1.1 1.1e-03]  MutualImpedance=[1.0 1.0e-03]  InductanceMatrix=Ll* L  ResistanceMatrix=Rl* L  Measurements=None
  Ground{2..3,5..6} (4 alike) : spsGroundLib/Ground  LConnTagsString=a
  Series RLC Branch : spsSeriesRLCBranchLib/Series RLC Branch  LConnTagsString=__new0  RConnTagsString=__new0  BranchType=C  Resistance=1  Inductance=1e-3  SetiL0=off  InitialCurrent=0  Capacitance=Cl(1,2)/2*L  Setx0=off  InitialVoltage=0  Measurements=None
  Series RLC Branch1 : spsSeriesRLCBranchLib/Series RLC Branch  LConnTagsString=__new0  RConnTagsString=__new0  BranchType=C  Resistance=1  Inductance=1e-3  SetiL0=off  InitialCurrent=0  Capacitance=Cl(1,2)/2*L  Setx0=off  InitialVoltage=0  Measurements=None
  Series RLC Branch11 : spsSeriesRLCBranchLib/Series RLC Branch  LConnTagsString=__new0  RConnTagsString=__new0  BranchType=C  Resistance=1  Inductance=1e-3  SetiL0=off  InitialCurrent=0  Capacitance=Cl(1,1)/2*L  Setx0=off  InitialVoltage=0  Measurements=None
  Series RLC Branch2 : spsSeriesRLCBranchLib/Series RLC Branch  LConnTagsString=__new0  RConnTagsString=__new0  BranchType=C  Resistance=1  Inductance=1e-3  SetiL0=off  InitialCurrent=0  Capacitance=Cl(1,1)/2*L  Setx0=off  InitialVoltage=0  Measurements=None
  Series RLC Branch3 : spsSeriesRLCBranchLib/Series RLC Branch  LConnTagsString=__new0  RConnTagsString=__new0  BranchType=C  Resistance=1  Inductance=1e-3  SetiL0=off  InitialCurrent=0  Capacitance=Cl(2,2)/2*L  Setx0=off  InitialVoltage=0  Measurements=None
  Series RLC Branch9 : spsSeriesRLCBranchLib/Series RLC Branch  LConnTagsString=__new0  RConnTagsString=__new0  BranchType=C  Resistance=1  Inductance=1e-3  SetiL0=off  InitialCurrent=0  Capacitance=Cl(2,2)/2*L  Setx0=off  InitialVoltage=0  Measurements=None
  B In : PMIOPort  Side=Left
  C in : PMIOPort  Port=2  Side=Left
  B Out : PMIOPort  Port=3  Side=Right
  C Out : PMIOPort  Port=4  Side=Right
  connections:
  Series RLC Branch2/RConn1 -- Ground2/LConn1
  Series RLC Branch3/RConn1 -- Ground5/LConn1
  Ground6/LConn1 -- Series RLC Branch9/RConn1
  Ground3/LConn1 -- Series RLC Branch11/RConn1
  C Out/RConn1 -- Series RLC Branch1/RConn1 -- Series RLC Branch3/LConn1 -- Config300/RConn2
  C in/RConn1 -- Series RLC Branch/RConn1 -- Series RLC Branch9/LConn1 -- Config300/LConn2
  B Out/RConn1 -- Series RLC Branch1/LConn1 -- Series RLC Branch2/LConn1 -- Config300/RConn1
  Series RLC Branch11/LConn1 -- B In/RConn1 -- Series RLC Branch/LConn1 -- Config300/LConn1

== system IEEE13_DVR_DSTATCOM_PV_Wind/646 ==
  1 : spsThreePhaseVIMeasurementLib/Three-Phase V-I Measurement  VoltageMeasurement=phase-to-ground  SetLabelV=on  LabelV=V646  Vpu=off  VpuLL=off  CurrentMeasurement=no  SetLabelI=on  LabelI=I634  Ipu=off  Pbase=100e6  Vbase=24900  OutputType=Complex  PhasorSimulation=off  PSBequivalent=0
  Ground12 : spsGroundLib/Ground  LConnTagsString=a
  Ground9 : spsGroundLib/Ground  LConnTagsString=a
  B : PMIOPort  Side=Right
  b : PMIOPort  Port=2  Side=Left
  c : PMIOPort  Port=3  Side=Left
  C : PMIOPort  Port=4  Side=Right
  connections:
  1/RConn3 -- c/RConn1
  1/RConn2 -- b/RConn1
  Ground9/LConn1 -- 1/RConn1
  1/LConn2 -- B/RConn1
  1/LConn3 -- C/RConn1
  Ground12/LConn1 -- 1/LConn1

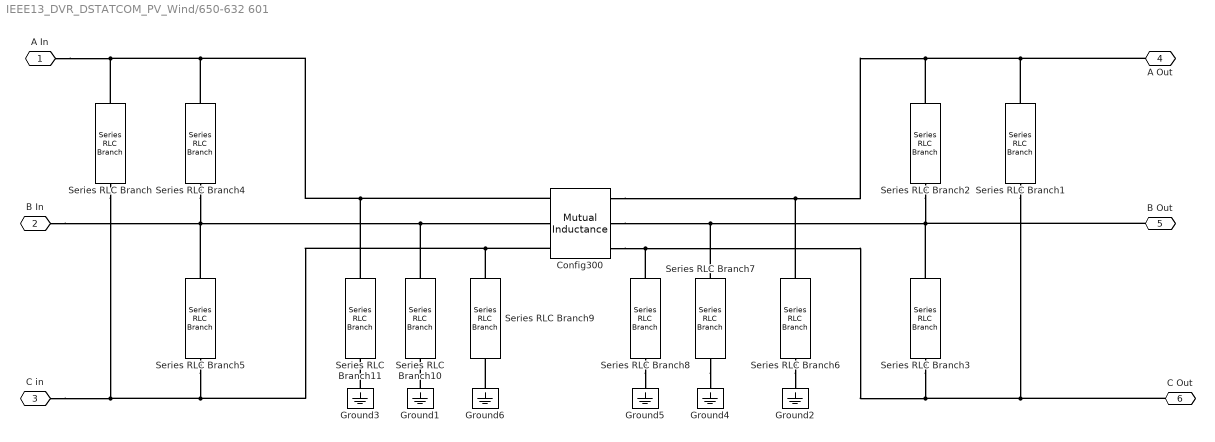
== system IEEE13_DVR_DSTATCOM_PV_Wind/650-632 601 ==
  Config300 : spsMutualInductanceLib/Mutual Inductance  LConnTagsString=a|b|c  RConnTagsString=A|B|C  TypeOfMutual=Generalized mutual inductance  NumberOfWindings=3  SelfImpedance1=[1.1 1.1e-03]  SelfImpedance2=[ 1.1 1.1e-03]  ThreeWindings=on  SelfImpedance3=[ 1.1 1.1e-03]  MutualImpedance=[1.0 1.0e-03]  InductanceMatrix=Ll* L  ResistanceMatrix=Rl* L  Measurements=None
  Ground{1..6} (6 alike) : spsGroundLib/Ground  LConnTagsString=a
  Series RLC Branch : spsSeriesRLCBranchLib/Series RLC Branch  LConnTagsString=__new0  RConnTagsString=__new0  BranchType=C  Resistance=1  Inductance=1e-3  SetiL0=off  InitialCurrent=0  Capacitance=Cl(1,3)/2*L  Setx0=off  InitialVoltage=0  Measurements=None
  Series RLC Branch1 : spsSeriesRLCBranchLib/Series RLC Branch  LConnTagsString=__new0  RConnTagsString=__new0  BranchType=C  Resistance=1  Inductance=1e-3  SetiL0=off  InitialCurrent=0  Capacitance=Cl(1,3)/2*L  Setx0=off  InitialVoltage=0  Measurements=None
  Series RLC Branch10 : spsSeriesRLCBranchLib/Series RLC Branch  LConnTagsString=__new0  RConnTagsString=__new0  BranchType=C  Resistance=1  Inductance=1e-3  SetiL0=off  InitialCurrent=0  Capacitance=Cl(2,2)/2*L  Setx0=off  InitialVoltage=0  Measurements=None
  Series RLC Branch11 : spsSeriesRLCBranchLib/Series RLC Branch  LConnTagsString=__new0  RConnTagsString=__new0  BranchType=C  Resistance=1  Inductance=1e-3  SetiL0=off  InitialCurrent=0  Capacitance=Cl(1,1)/2*L  Setx0=off  InitialVoltage=0  Measurements=None
  Series RLC Branch2 : spsSeriesRLCBranchLib/Series RLC Branch  LConnTagsString=__new0  RConnTagsString=__new0  BranchType=C  Resistance=1  Inductance=1e-3  SetiL0=off  InitialCurrent=0  Capacitance=Cl(1,2)/2*L  Setx0=off  InitialVoltage=0  Measurements=None
  Series RLC Branch3 : spsSeriesRLCBranchLib/Series RLC Branch  LConnTagsString=__new0  RConnTagsString=__new0  BranchType=C  Resistance=1  Inductance=1e-3  SetiL0=off  InitialCurrent=0  Capacitance=Cl(2,3)/2*L  Setx0=off  InitialVoltage=0  Measurements=None
  Series RLC Branch4 : spsSeriesRLCBranchLib/Series RLC Branch  LConnTagsString=__new0  RConnTagsString=__new0  BranchType=C  Resistance=1  Inductance=1e-3  SetiL0=off  InitialCurrent=0  Capacitance=Cl(1,2)/2*L  Setx0=off  InitialVoltage=0  Measurements=None
  Series RLC Branch5 : spsSeriesRLCBranchLib/Series RLC Branch  LConnTagsString=__new0  RConnTagsString=__new0  BranchType=C  Resistance=1  Inductance=1e-3  SetiL0=off  InitialCurrent=0  Capacitance=Cl(2,3)/2*L  Setx0=off  InitialVoltage=0  Measurements=None
  Series RLC Branch6 : spsSeriesRLCBranchLib/Series RLC Branch  LConnTagsString=__new0  RConnTagsString=__new0  BranchType=C  Resistance=1  Inductance=1e-3  SetiL0=off  InitialCurrent=0  Capacitance=Cl(1,1)/2*L  Setx0=off  InitialVoltage=0  Measurements=None
  Series RLC Branch7 : spsSeriesRLCBranchLib/Series RLC Branch  LConnTagsString=__new0  RConnTagsString=__new0  BranchType=C  Resistance=1  Inductance=1e-3  SetiL0=off  InitialCurrent=0  Capacitance=Cl(2,2)/2*L  Setx0=off  InitialVoltage=0  Measurements=None
  Series RLC Branch8 : spsSeriesRLCBranchLib/Series RLC Branch  LConnTagsString=__new0  RConnTagsString=__new0  BranchType=C  Resistance=1  Inductance=1e-3  SetiL0=off  InitialCurrent=0  Capacitance=Cl(3,3)/2*L  Setx0=off  InitialVoltage=0  Measurements=None
  Series RLC Branch9 : spsSeriesRLCBranchLib/Series RLC Branch  LConnTagsString=__new0  RConnTagsString=__new0  BranchType=C  Resistance=1  Inductance=1e-3  SetiL0=off  InitialCurrent=0  Capacitance=Cl(3,3)/2*L  Setx0=off  InitialVoltage=0  Measurements=None
  A In : PMIOPort  Side=Left
  B In : PMIOPort  Port=2  Side=Left
  C in : PMIOPort  Port=3  Side=Left
  A Out : PMIOPort  Port=4  Side=Right
  B Out : PMIOPort  Port=5  Side=Right
  C Out : PMIOPort  Port=6  Side=Right
  connections:
  Series RLC Branch6/RConn1 -- Ground2/LConn1
  Series RLC Branch7/RConn1 -- Ground4/LConn1
  Series RLC Branch8/RConn1 -- Ground5/LConn1
  Ground6/LConn1 -- Series RLC Branch9/RConn1
  Ground1/LConn1 -- Series RLC Branch10/RConn1
  Ground3/LConn1 -- Series RLC Branch11/RConn1
  C Out/RConn1 -- Series RLC Branch1/RConn1 -- Series RLC Branch3/RConn1 -- Series RLC Branch8/LConn1 -- Config300/RConn3
  C in/RConn1 -- Series RLC Branch/RConn1 -- Series RLC Branch5/RConn1 -- Series RLC Branch9/LConn1 -- Config300/LConn3
  A Out/RConn1 -- Series RLC Branch1/LConn1 -- Series RLC Branch2/LConn1 -- Series RLC Branch6/LConn1 -- Config300/RConn1
  A In/RConn1 -- Series RLC Branch/LConn1 -- Series RLC Branch4/LConn1 -- Series RLC Branch11/LConn1 -- Config300/LConn1
  B Out/RConn1 -- Series RLC Branch2/RConn1 -- Series RLC Branch3/LConn1 -- Series RLC Branch7/LConn1 -- Config300/RConn2
  B In/RConn1 -- Config300/LConn2 -- Series RLC Branch10/LConn1 -- Series RLC Branch5/LConn1 -- Series RLC Branch4/RConn1

== system IEEE13_DVR_DSTATCOM_PV_Wind/652 ==
  1 : spsThreePhaseVIMeasurementLib/Three-Phase V-I Measurement  VoltageMeasurement=phase-to-ground  SetLabelV=on  LabelV=V652  Vpu=off  VpuLL=off  CurrentMeasurement=no  SetLabelI=on  LabelI=I634  Ipu=off  Pbase=100e6  Vbase=24900  OutputType=Complex  PhasorSimulation=off  PSBequivalent=0
  Ground{1..2,9,12} (4 alike) : spsGroundLib/Ground  LConnTagsString=a
  a : PMIOPort  Side=Left
  A : PMIOPort  Port=2  Side=Right
  connections:
  Ground9/LConn1 -- 1/RConn2
  Ground12/LConn1 -- 1/LConn2
  Ground2/LConn1 -- 1/LConn3
  Ground1/LConn1 -- 1/RConn3
  A/RConn1 -- 1/LConn1
  a/RConn1 -- 1/RConn1

== system IEEE13_DVR_DSTATCOM_PV_Wind/671-684 604 ==
  Config300 : spsMutualInductanceLib/Mutual Inductance  LConnTagsString=a|b  RConnTagsString=A|B  TypeOfMutual=Generalized mutual inductance  NumberOfWindings=2  SelfImpedance1=[1.1 1.1e-03]  SelfImpedance2=[ 1.1 1.1e-03]  ThreeWindings=on  SelfImpedance3=[ 1.1 1.1e-03]  MutualImpedance=[1.0 1.0e-03]  InductanceMatrix=Ll* L  ResistanceMatrix=Rl* L  Measurements=None
  Ground{2..3,5..6} (4 alike) : spsGroundLib/Ground  LConnTagsString=a
  Series RLC Branch : spsSeriesRLCBranchLib/Series RLC Branch  LConnTagsString=__new0  RConnTagsString=__new0  BranchType=C  Resistance=1  Inductance=1e-3  SetiL0=off  InitialCurrent=0  Capacitance=Cl(1,2)/2*L  Setx0=off  InitialVoltage=0  Measurements=None
  Series RLC Branch1 : spsSeriesRLCBranchLib/Series RLC Branch  LConnTagsString=__new0  RConnTagsString=__new0  BranchType=C  Resistance=1  Inductance=1e-3  SetiL0=off  InitialCurrent=0  Capacitance=Cl(1,2)/2*L  Setx0=off  InitialVoltage=0  Measurements=None
  Series RLC Branch11 : spsSeriesRLCBranchLib/Series RLC Branch  LConnTagsString=__new0  RConnTagsString=__new0  BranchType=C  Resistance=1  Inductance=1e-3  SetiL0=off  InitialCurrent=0  Capacitance=Cl(1,1)/2*L  Setx0=off  InitialVoltage=0  Measurements=None
  Series RLC Branch2 : spsSeriesRLCBranchLib/Series RLC Branch  LConnTagsString=__new0  RConnTagsString=__new0  BranchType=C  Resistance=1  Inductance=1e-3  SetiL0=off  InitialCurrent=0  Capacitance=Cl(1,1)/2*L  Setx0=off  InitialVoltage=0  Measurements=None
  Series RLC Branch3 : spsSeriesRLCBranchLib/Series RLC Branch  LConnTagsString=__new0  RConnTagsString=__new0  BranchType=C  Resistance=1  Inductance=1e-3  SetiL0=off  InitialCurrent=0  Capacitance=Cl(2,2)/2*L  Setx0=off  InitialVoltage=0  Measurements=None
  Series RLC Branch9 : spsSeriesRLCBranchLib/Series RLC Branch  LConnTagsString=__new0  RConnTagsString=__new0  BranchType=C  Resistance=1  Inductance=1e-3  SetiL0=off  InitialCurrent=0  Capacitance=Cl(2,2)/2*L  Setx0=off  InitialVoltage=0  Measurements=None
  A In : PMIOPort  Side=Left
  C in : PMIOPort  Port=2  Side=Left
  A Out : PMIOPort  Port=3  Side=Right
  C Out : PMIOPort  Port=4  Side=Right
  connections:
  Series RLC Branch2/RConn1 -- Ground2/LConn1
  Series RLC Branch3/RConn1 -- Ground5/LConn1
  Ground6/LConn1 -- Series RLC Branch9/RConn1
  Ground3/LConn1 -- Series RLC Branch11/RConn1
  Series RLC Branch3/LConn1 -- Config300/RConn2 -- C Out/RConn1 -- Series RLC Branch1/RConn1
  C in/RConn1 -- Series RLC Branch/RConn1 -- Series RLC Branch9/LConn1 -- Config300/LConn2
  Series RLC Branch2/LConn1 -- Config300/RConn1 -- A Out/RConn1 -- Series RLC Branch1/LConn1
  Series RLC Branch11/LConn1 -- A In/RConn1 -- Series RLC Branch/LConn1 -- Config300/LConn1

== system IEEE13_DVR_DSTATCOM_PV_Wind/680 ==
  1 : spsThreePhaseVIMeasurementLib/Three-Phase V-I Measurement  VoltageMeasurement=phase-to-ground  SetLabelV=on  LabelV=V680  Vpu=off  VpuLL=off  CurrentMeasurement=yes  SetLabelI=on  LabelI=I680  Ipu=off  Pbase=100e6  Vbase=24900  OutputType=Complex  PhasorSimulation=off  PSBequivalent=0
  A : PMIOPort  Side=Right
  B : PMIOPort  Port=2  Side=Right
  C : PMIOPort  Port=3  Side=Right
  connections:
  1/LConn1 -- A/RConn1
  1/LConn2 -- B/RConn1
  C/RConn1 -- 1/LConn3

== system IEEE13_DVR_DSTATCOM_PV_Wind/684 ==
  1 : spsThreePhaseVIMeasurementLib/Three-Phase V-I Measurement  VoltageMeasurement=phase-to-ground  SetLabelV=on  LabelV=V684  Vpu=off  VpuLL=off  CurrentMeasurement=no  SetLabelI=on  LabelI=I634  Ipu=off  Pbase=100e6  Vbase=24900  OutputType=Complex  PhasorSimulation=off  PSBequivalent=0
  Ground12 : spsGroundLib/Ground  LConnTagsString=a
  Ground9 : spsGroundLib/Ground  LConnTagsString=a
  A : PMIOPort  Side=Right
  a : PMIOPort  Port=2  Side=Left
  c : PMIOPort  Port=3  Side=Left
  C : PMIOPort  Port=4  Side=Right
  connections:
  1/RConn3 -- c/RConn1
  1/LConn3 -- C/RConn1
  Ground9/LConn1 -- 1/RConn2
  a/RConn1 -- 1/RConn1
  Ground12/LConn1 -- 1/LConn2
  1/LConn1 -- A/RConn1

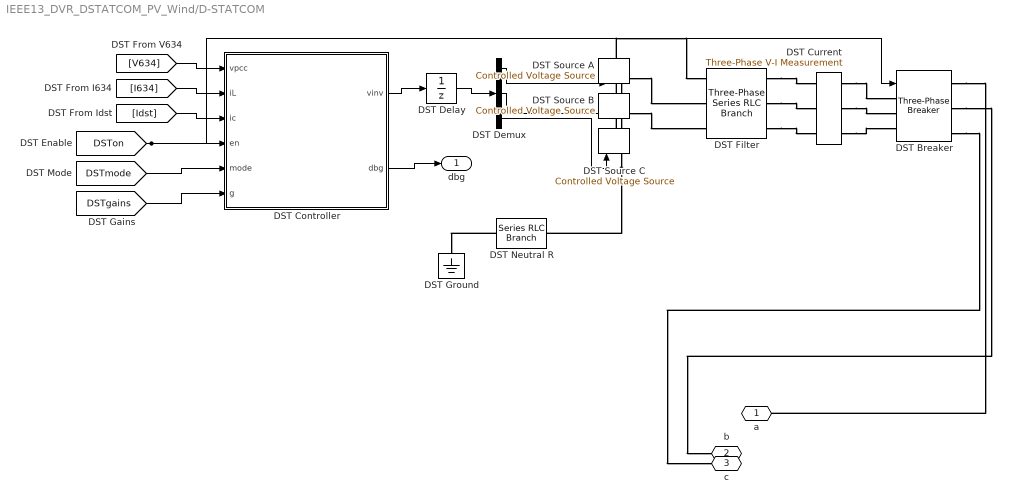
== system IEEE13_DVR_DSTATCOM_PV_Wind/D-STATCOM ==
  DST Breaker : spsThreePhaseBreakerLib/Three-Phase Breaker  InitialState=open  SwitchA=on  SwitchB=on  SwitchC=on  SwitchTimes=[0.4]  External=on  BreakerResistance=0.01  SnubberResistance=1e6  SnubberCapacitance=inf  Measurements=None
  DST Controller : MATLAB Function  TreatAsAtomicUnit=on
  DST Current : spsThreePhaseVIMeasurementLib/Three-Phase V-I Measurement  VoltageMeasurement=no  SetLabelV=off  LabelV=Vabc  Vpu=off  VpuLL=off  CurrentMeasurement=yes  SetLabelI=on  LabelI=Idst  Ipu=off  Pbase=100e6  Vbase=500e3  OutputType=Complex  PhasorSimulation=off  PSBequivalent=0
  DST Delay : UnitDelay  SampleTime=-1  HasFrameUpgradeWarning=on
  DST Demux : Demux  Outputs=3
  DST Filter : spsThreePhaseSeriesRLCBranchLib/Three-Phase Series RLC Branch  LConnTagsString=A|B|C  RConnTagsString=A|B|C  BranchType=RL  Resistance=5e-3  Inductance=0.2e-3  Capacitance=1e-6  Measurements=None
  DST Ground : spsGroundLib/Ground  LConnTagsString=a
  DST Neutral R : spsSeriesRLCBranchLib/Series RLC Branch  LConnTagsString=__new0  RConnTagsString=__new0  BranchType=R  Resistance=1e6  Inductance=1e-3  SetiL0=off  InitialCurrent=0  Capacitance=1e-6  Setx0=off  InitialVoltage=0  Measurements=None
  DST Source A : spsControlledVoltageSourceLib/Controlled Voltage Source  Initialize=off  Source_Type=AC  Amplitude=0  Phase=0  Frequency=0  Measurements=None
  DST Source B : spsControlledVoltageSourceLib/Controlled Voltage Source  Initialize=off  Source_Type=AC  Amplitude=0  Phase=0  Frequency=0  Measurements=None
  DST Source C : spsControlledVoltageSourceLib/Controlled Voltage Source  Initialize=off  Source_Type=AC  Amplitude=0  Phase=0  Frequency=0  Measurements=None
  a : PMIOPort  Side=Right
  b : PMIOPort  Port=2  Side=Right
  c : PMIOPort  Port=3  Side=Right
  dbg : Outport
  wires:
  [V634] -> DST Controller/1(vpcc)
  DST Controller/2(dbg) -> dbg/1
  DST Demux/2 -> DST Source B/1
  [I634] -> DST Controller/2(iL)
  DST Controller/1(vinv) -> DST Delay/1
  [Idst] -> DST Controller/3(ic)
  DST Delay/1 -> DST Demux/1
  DST Demux/1 -> DST Source A/1
  DST Demux/3 -> DST Source C/1
  [DSTon] -> DST Controller/4(en), DST Breaker/1
  [DSTmode] -> DST Controller/5(mode)
  [DSTgains] -> DST Controller/6(g)
  connections:
  DST Breaker/RConn1 -- a/RConn1
  DST Source A/LConn1 -- DST Neutral R/RConn1 -- DST Source C/LConn1 -- DST Source B/LConn1
  DST Filter/RConn1 -- DST Current/LConn1
  DST Current/RConn3 -- DST Breaker/LConn3
  DST Neutral R/LConn1 -- DST Ground/LConn1
  DST Filter/RConn2 -- DST Current/LConn2
  DST Source C/RConn1 -- DST Filter/LConn3
  DST Current/RConn2 -- DST Breaker/LConn2
  DST Source A/RConn1 -- DST Filter/LConn1
  DST Current/RConn1 -- DST Breaker/LConn1
  DST Filter/RConn3 -- DST Current/LConn3
  DST Source B/RConn1 -- DST Filter/LConn2
  DST Breaker/RConn3 -- c/RConn1
  DST Breaker/RConn2 -- b/RConn1
